simulink model "hdlFrame_FogRectification_3D_MLFB"  (R2025b)
settings: Solver=FixedStepDiscrete  StopTime=3  EnableMultiTasking=on
InitFcn:
  | thresh=.0015;
  | d5 = [-1 8 0 -8 1]/12;
  | p5 = [1 4 6 4 1]/16;
  | b = ones(1,5)/5;
  | Angle = 98.39185;
  | InitialConditon = 0;
  | line_row = 22;
  | sz = 50;
model workspace (MAT data in the model file):
  SourceMovingObject = 0
  gainValueHSV = 0.2
libraries: visionsources x1
settings Model: Creator=abehbood  LastModifiedBy=jmazur
settings SolverCC: AlgebraicLoopSolver=TrustRegion  MaxZcPerStep=1.0
settings DataIOCC: ReturnWorkspaceOutputs=off
settings OptimizationCC: BlockReduction=off  ConditionallyExecuteInputs=off  EfficientMapNaN2IntZero=off  LifeSpan=inf
settings DebuggingCC: SignalRangeChecking=warning  UnconnectedInputMsg=warning  UnconnectedOutputMsg=warning  UnconnectedLineMsg=warning  SFUnexpectedBacktrackingDiag=warning  SFNoUnconditionalDefaultTransitionDiag=warning  ArithmeticOperatorsInVariantConditions=warning
settings HardwareCC: TargetBitPerLong=64.0  TargetBitPerPointer=64.0  TargetBitPerSizeT=64.0  TargetBitPerPtrDiffT=64.0  TargetLongLongMode=on  TargetIntDivRoundTo=Zero  TargetEndianess=LittleEndian  TargetWordSize=64.0  TargetHWDeviceType=MATLAB Host  ProdEqTarget=off
settings ModelReferenceCC: EnableRefExpFcnMdlSchedulingChecks=on
settings SFSimCC: SimUseLocalCustomCode=off  CustomCodeUndefinedFunction=UseInterfaceOnly
settings RTWCC: RTWUseLocalCustomCode=off  GPUComputeCapability=3.5  DLArmComputeVersion=19.05
settings CodeAppCC: MaxIdLength=128.0  StateflowObjectComments=on
settings GRTTargetCC: TargetLangStandard=C89/C90 (ANSI)  CombineOutputUpdateFcns=off  GRTInterface=on
settings ConfigComp: CovMetricSettings=dw  CovSaveCumulativeToWorkspaceVar=on  CovSaveSingleToWorkspaceVar=on  CovExternalEMLEnable=off

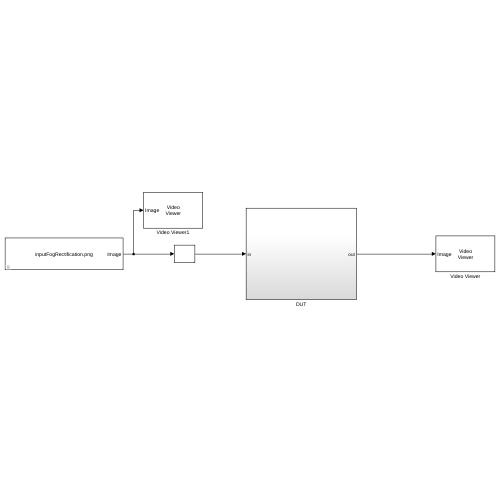
[thumbnail: Simulink's stored preview of the top-level diagram]
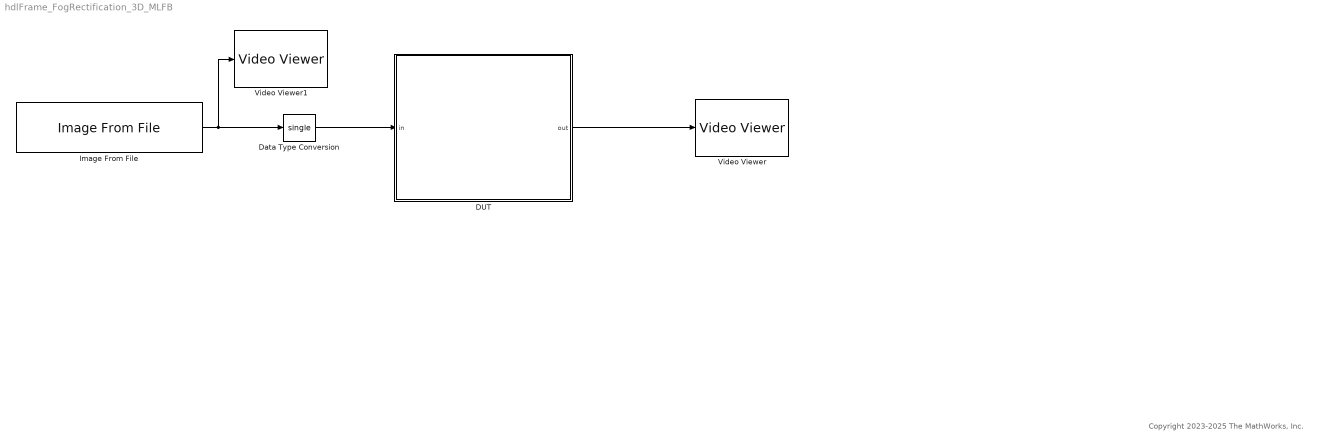
== system hdlFrame_FogRectification_3D_MLFB ==
  note: Copyright 2023-2025 The MathWorks, Inc.
  DUT : Subsystem
  Data Type Conversion : DataTypeConversion  OutDataTypeStr=single  SaturateOnIntegerOverflow=off  RndMeth=Floor
  Image From File : visionsources/Image From File  Tag=vipblks_nd  FileName=inputFogRectification.png  Ts=1  imagePorts=One multidimensional signal  OutPortLabels=R|G|B  ImageDataType=uint8  sdImageDataType=uint(8)  Signed=on  WordLength=16  FractionLengthMode=User-defined  FractionLength=15
  Video Viewer : VideoViewer  FigPos=[1437.66666666667 861 313.33333333333 211]
  Video Viewer1 : VideoViewer  FigPos=[1428.33333333333 557.333333333333 412 301.333333333333]
  wires:
  DUT/1(out) -> Video Viewer/1
  Data Type Conversion/1 -> DUT/1(in)
  Image From File/1 -> Video Viewer1/1, Data Type Conversion/1

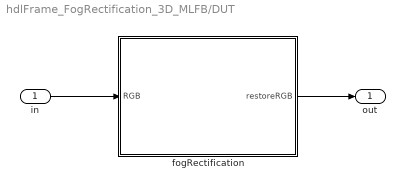
== system hdlFrame_FogRectification_3D_MLFB/DUT ==
  in : Inport
  fogRectification : MATLAB Function  TreatAsAtomicUnit=on
  out : Outport
  wires:
  fogRectification/1(restoreRGB) -> out/1
  in/1 -> fogRectification/1(RGB)

== matlab function hdlFrame_FogRectification_3D_MLFB/DUT/fogRectification ==
  settings: fimath=hdlfimath
  data: RGB input; restoreRGB output
function restoreRGB = fogRectification(RGB)

R = RGB(:,:,1);
G = RGB(:,:,2);
B = RGB(:,:,3);

% Changing the precision level of input image to double
R = R / 255;
G = G / 255;
B = B / 255;

%% Dark channel Estimation from input
darkChannel = hdl.npufun(@min_kernel, [1 1], R, G, B);

% diff_im is used as input and output variable for anisotropic diffusion
diff_im = 0.9*darkChannel;

%% Refine dark channel using Anisotropic diffusion.
diff_im = hdl.npufun(@filter_kernel, [3 3], diff_im);
diff_im = hdl.npufun(@filter_kernel, [3 3], diff_im);
diff_im = hdl.npufun(@filter_kernel, [3 3], diff_im);

%% Reduction with min
% diff_im = min(darkChannel,diff_im);
diff_im = hdl.npufun(@min_kernel2, [1 1], darkChannel, diff_im);

diff_im = 0.6*diff_im ;

%% Parallel element-wise math to compute
%  Restoration with inverse Koschmieder's law
factor = 1.0./(1.0-(diff_im));
restoreRs = (R-diff_im).*factor;
restoreGs = (G-diff_im).*factor;
restoreBs = (B-diff_im).*factor;

% Convert to integer
restoreR = uint8(255.*restoreRs);
restoreG = uint8(255.*restoreGs);
restoreB = uint8(255.*restoreBs);

%%
% Stretching performs the histogram stretching of the image.
% im is the input color image and p is cdf limit.
% out is the contrast stretched image and cdf is the cumulative prob.
% density function and T is the stretching function.
% RGB to grayscale conversion
im_gray = hdl.npufun(@convert_gray, [1 1], restoreR, restoreG, restoreB);

% [restoreR, restoreG, restoreB] = hdl.npufun(@zero_to_one, [1 1], restoreR, restoreG, restoreB);
% restoreR(restoreR == 0) = 1;
% restoreG(restoreG == 0) = 1;
% restoreB(restoreB == 0) = 1;

% Rewriting 0-1 setting to avoid reshape
zeros_to_one = (restoreR == 0);
restoreR = restoreR + uint8(zeros_to_one);
zeros_to_one = (restoreG == 0);
restoreG = restoreG + uint8(zeros_to_one);
zeros_to_one = (restoreR == 0);
restoreB = restoreB + uint8(zeros_to_one);


[r_out,g_out,b_out] = fog_rectification_stage2(im_gray, restoreR, restoreG, restoreB);

restoreRGB = cat(3, r_out,g_out,b_out);

end

function out = filter_kernel(in)
hN = single([0.0625 0.1250 0.0625; 0.1250 0.2500 0.1250; 0.0625 0.1250 0.0625]);
out = sum(in(:).*hN(:), 'native');
end

function out = min_kernel(R, G, B)
    out = min([R, G, B]);
end

function out = convert_gray(R, G, B)

out = uint8(round(0.2989 * single(R) + 0.5870 * single(G) + 0.1140 * single(B)));

end

function out = min_kernel2(A, B)
    out = min(A, B);
end


function [r_out,g_out,b_out] = fog_rectification_stage2(im_gray, r, g, b)
%FOG_RECTIFICATION_HDL_3_STAGE2 
% histogram computation
% Find cdf
% Find breakpoints of table
% Compute table
% Use table on input image to create output image

% histogram calculation
hist = zeros(1, 256, 'uint32');
hist = reduce(@hist_kernel_fcn, im_gray, hist);

% cumulative Sum calculation
% cdf=cumsum(prob(:));
cdf = zeros(256,1,'uint32');
coder.hdl.loopspec('stream');
for ii=int32(1:numel(hist))
    prob = hist(ii); % normalize
    if ii > 1
        cdf(ii) = cdf(ii-1) + prob;
    else
        cdf(1) = prob;
    end
%     cdf(ii) = single(cdf(ii)*invSize);
end

% finding less than particular probability
% i1=length(find(cdf<=(p/100)));
% i2=255-length(find(cdf>=1-(p/100)));
N = numel(im_gray);
p1 = fi(5*N/100);
p2 = fi(N-(5*N/100));
i1 = uint8(0); i2 = uint8(0);
coder.hdl.loopspec('stream');
for it=int32(1:numel(cdf))
    if (cdf(it) <= p1)
        i1 = i1 + 1;
    end
    
    if (cdf(it) >= p2)
        i2 = i2 + 1;
    end
end
i2 = 255-i2;

% lookup table
o1 = single(255*0.10);
o2 = single(255*0.90);

t1 = o1/single(i1);
t2 = (o2-o1)/single(i2-i1);
t3 = (255-o2)/single(255-i2);

t1f = fi(t1, 0, 32, 24);
t2f = fi(t2, 0, 32, 24);
t3f = fi(t3, 0, 32, 24);

T = zeros(1,256, 'uint8');
coder.hdl.loopspec('stream');
for i = int32(1:256)
    is = uint8(i);
    if is <= i1+1
        T(i) = uint8(t1f*(is-1));
    elseif is >= i1+2 && is <= i2+1
        T(i) = uint8(((t2f)*(is-1))-((t2f)*i1)+o1);
    else
        T(i) = uint8(((t3f)*(is-1))-((t3f)*i2)+o2);
    end
end

r_out = coder.nullcopy(zeros(size(r), 'uint8'));
g_out = coder.nullcopy(zeros(size(r), 'uint8'));
b_out = coder.nullcopy(zeros(size(r), 'uint8'));
coder.hdl.loopspec('stream');
for it=int32(1:numel(r))

    out1=T(r(it));
    out2=T(g(it));
    out3=T(b(it));

    r_out(it) = uint8(out1);
    g_out(it) = uint8(out2);
    b_out(it) = uint8(out3);
end

end

function out = reduce(kernelFun, I, data)

%   Copyright 2021 The MathWorks, Inc.

assert(isa(kernelFun, 'function_handle'), ...
    'kernelFun must be a function handle');

coder.hdl.loopspec('stream');
for ii=int32(1:numel(I))
    data = kernelFun(I(ii), data);
end
out = data;

end

function count = hist_kernel_fcn(pix, count)

count(pix+1) = count(pix+1) +1;

end
